simulink model "Q5_2_4"  (R2023b)
settings: Solver=ode45  StartTime=0.0  StopTime=15.0  RelTol=1e-3
settings Model: Creator=Arshia  LastModifiedBy=Arshia

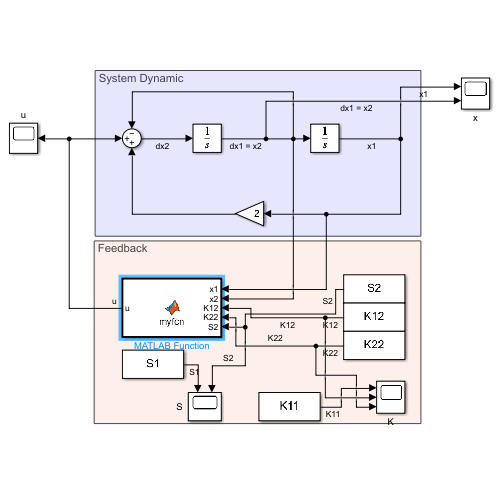
[thumbnail: Simulink's stored preview of the top-level diagram]
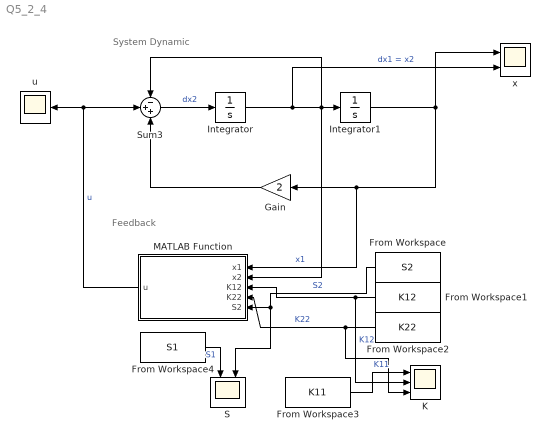
== system Q5_2_4 ==
  note: Feedback
  note: System Dynamic
  From Workspace : FromWorkspace  VariableName=S2
  From Workspace1 : FromWorkspace  VariableName=K12
  From Workspace2 : FromWorkspace  VariableName=K22
  From Workspace3 : FromWorkspace  VariableName=K11
  From Workspace4 : FromWorkspace  VariableName=S1
  Gain : Gain  Gain=2
  Integrator : Integrator
  Integrator1 : Integrator  InitialCondition=-4
  K : Scope  NumInputPorts=3
  MATLAB Function : MATLAB Function  TreatAsAtomicUnit=on
  S : Scope  NumInputPorts=2
  Sum3 : Sum  Inputs=-++
  u : Scope
  x : Scope  NumInputPorts=2
  wires:
  From Workspace/1 -> S/2, MATLAB Function/5(S2)  "S2"
  From Workspace1/1 -> MATLAB Function/3(K12), K/2  "K12"
  MATLAB Function/1(u) -> Sum3/2, u/1  "u"
  From Workspace2/1 -> MATLAB Function/4(K22), K/3  "K22"
  Sum3/1 -> Integrator/1  "dx2"
  Gain/1 -> Sum3/3
  Integrator/1 -> x/2, Sum3/1, MATLAB Function/2(x2), Integrator1/1  "dx1 = x2"
  Integrator1/1 -> MATLAB Function/1(x1), Gain/1, x/1  "x1"
  From Workspace3/1 -> K/1  "K11"
  From Workspace4/1 -> S/1  "S1"

== matlab function Q5_2_4/MATLAB Function ==
  data: u output; x1 input; x2 input; K12 input; K22 input; S2 input
function u =myfcn(x1,x2,K12,K22,S2)
u=-20*(K12*x1 + K22*x2 + S2);
end
